simulink model "sim_closed_loop_with_identifiedmodel"  (R2024a)
settings: Solver=FixedStepAuto  StartTime=0.0  StopTime=10  FixedStep=1/fs  RelTol=1e-3
PostLoadFcn:
  | if any(exist('dsrtsu_mdlpostloadfcn', 'file') ~= 0), dsrtsu_mdlpostloadfcn('Execute', bdroot); end
InitFcn:
  | , if any(exist('rtifpga_mdlclblib', 'file') ~= 0), rtifpga_mdlclblib('Init', bdroot); end,
  | , if any(exist('dsmpb_private', 'file') ~= 0), dsmpb_private('dsmpb_mdlclblib', 'Init', bdroot); end,
values from neighbouring files (symbols this model uses):
  fcut = 2    [Fig09_compute_Xcorr_CLID.m]
  fs = 2000    [Fig09_compute_Xcorr_CLID.m]    (also in Fig10_compare_ID_closedloop.m)
  KdDMD = dlqr(Akdmd, Bkdmd, Qkdmd, 1)    [Fig09_compute_Xcorr_CLID.m]
  nuf = size(Bf,2)    [Fig09_compute_Xcorr_CLID.m]
  nxf = size(Af,1)    [Fig09_compute_Xcorr_CLID.m]
  sysID2 = sysID    [Fig09_compute_Xcorr_CLID.m]
  x0 = zeros(nzeta,1)    [Fig09_compute_Xcorr_CLID.m]
undefined symbols (not defined in the file or in its folder): Af, Bf
libraries: dspfdesign x1
PreSaveFcn:
  | , if any(exist('dsmpb_private', 'file') ~= 0), dsmpb_private('dsmpb_mdlclblib', 'PreSave', bdroot); end,
CloseFcn:
  | , if any(exist('dsmpb_private', 'file') ~= 0), dsmpb_private('dsmpb_mdlclblib', 'Close', bdroot); end,
settings Model: DSRTSU_INTERNAL_RTI_VER=570  DSRTSU_INTERNAL_RTI_TYPE=rti1202  RTICANMMDATA=struct('GeneralSetupData',struct('modelroot',['C:\Users\fthais\Desktop\Fernanda 03-25\Matlab - Simulink\10-07'],'generalsettings',struct('filesettings',struct('destfolder',struct('Name','RTICANMM_FILES','Check',1),'buildfolder',struct('Name','.','Check',1),'AbsDestfolder',struct('Name',['C:\Users\fthais\Desktop\Fernanda 03-25\Matlab - Simulink\10-07\RTICANMM_FILES']),'AbsBuildfolder',struct('Name',['C:\Users\fthais\Desktop\Fernanda 03-25\Matlab - Simulink\10-07']))),'options',struct('addpaths',1,'rmpaths',1,'addtrcexclusion',true,'cannavigator',struct('checkmonitoring',0),'show_usrtrc',0,'use_usrtrc',0),'advanced',struct('options',ones(1,100)),'MPSetup',{{}},'RTI',struct('Type','RTI1202','Ver','7.15','Date','02-Nov-2020'),'modelname','comm_beam','block','comm_beam'))  DSRTSU_INTERNAL_RTIFPGA=170  Creator=ADP-sletellier  LastModifiedBy=fertc
settings SolverCC: AlgebraicLoopSolver=TrustRegion
settings OptimizationCC: BlockReduction=off  ConditionallyExecuteInputs=off  OptimizeBlockIOStorage=off  BufferReuse=off  GlobalBufferReuse=off  ExpressionFolding=off  LocalBlockOutputs=off  OptimizeDataStoreBuffers=off  BusAssignmentInplaceUpdate=off
settings DebuggingCC: TasksWithSamePriorityMsg=none  UnconnectedInputMsg=warning  UnconnectedOutputMsg=warning  UnconnectedLineMsg=warning
settings HardwareCC: ProdBitPerPointer=32  ProdBitPerSizeT=32  ProdBitPerPtrDiffT=32  ProdLargestAtomicInteger=Integer  ProdEndianess=BigEndian  ProdWordSize=32  ProdLongLongMode=on  ProdHWDeviceType=Custom Processor->Custom  TargetIntDivRoundTo=Zero  TargetEndianess=BigEndian  TargetHWDeviceType=Custom Processor->Custom
settings ModelReferenceCC: EnableRefExpFcnMdlSchedulingChecks=on  EnableParallelModelReferenceBuilds=on
settings SFSimCC: MATLABDynamicMemAlloc=off
settings RTWCC: Description=dSPACE DS1202 Hardware Platform  SystemTargetFile=rti1202.tlc  GenCodeOnly=on  MakeCommand=make_rti  TemplateMakefile=rti1202.tmf  RTWVerbose=off  GPUComputeCapability=3.5
settings STFCustomTargetCC: TargetLangStandard=C89/C90 (ANSI)  ParMdlRefBuildCompliant=on  GRTInterface=off  UseToolchainInfoCompliant=off  SystemTargetFile=rti1202.tlc
settings GRTTargetCC: TargetLangStandard=C89/C90 (ANSI)  CompOptLevelCompliant=off  ConcurrentExecutionCompliant=off  CombineOutputUpdateFcns=off  MatFileLogging=off  CPPClassGenCompliant=off  UseToolchainInfoCompliant=off

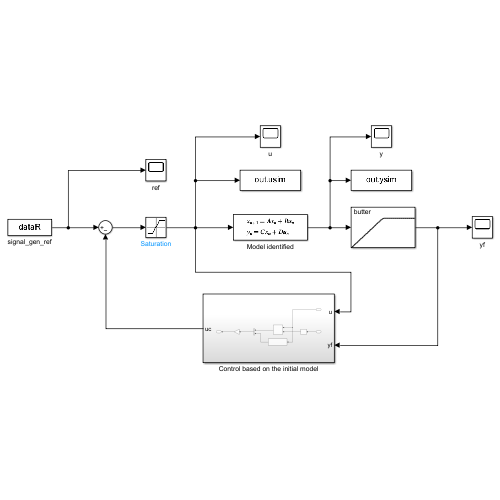
[thumbnail: Simulink's stored preview of the top-level diagram]
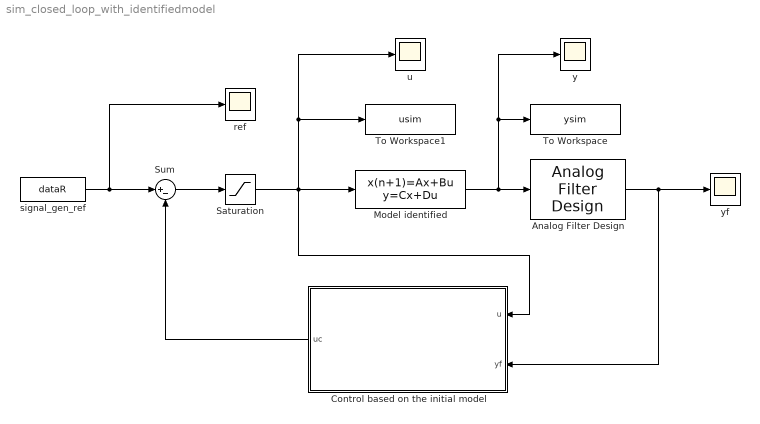
== system sim_closed_loop_with_identifiedmodel ==
  Analog Filter Design : dspfdesign/Analog Filter Design  method=Butterworth  filttype=Highpass  N=8  Wlo=2*pi*fcut  Whi=80  Rp=2  Rs=40
  Control based on the initial model : Subsystem
  Model identified : DiscreteStateSpace  A=sysID2.A  B=sysID2.B  C=sysID2.C  D=sysID2.D  SampleTime=1/fs
  Saturation : Saturate  UpperLimit=10  LowerLimit=-10
  Sum : Sum  Inputs=|+-
  To Workspace : ToWorkspace  VariableName=ysim  SaveFormat=Timeseries  SampleTime=-1
  To Workspace1 : ToWorkspace  VariableName=usim  SaveFormat=Timeseries  SampleTime=-1
  ref : Scope
  signal_gen_ref : FromWorkspace  VariableName=dataR  SampleTime=1/fs  Interpolate=off  OutputAfterFinalValue=Setting to zero
  u : Scope
  y : Scope
  yf : Scope
  wires:
  Analog Filter Design/1 -> yf/1, Control based on the initial model/2(yf)
  Saturation/1 -> Model identified/1, u/1, To Workspace1/1, Control based on the initial model/1(u)
  signal_gen_ref/1 -> ref/1, Sum/1
  Sum/1 -> Saturation/1
  Model identified/1 -> y/1, To Workspace/1, Analog Filter Design/1
  Control based on the initial model/1(uc) -> Sum/2

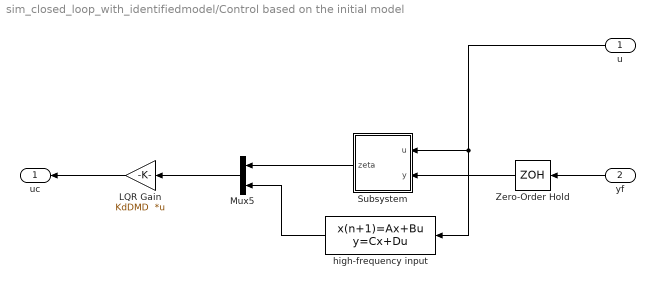
== system sim_closed_loop_with_identifiedmodel/Control based on the initial model ==
  u : Inport
  yf : Inport  Port=2
  LQR Gain : Gain  Gain=KdDMD  Multiplication=Matrix(K*u)
  Mux5 : Mux  Inputs=2
  Subsystem : Subsystem
  Zero-Order Hold : ZeroOrderHold  SampleTime=1/fs
  high-frequency input : DiscreteStateSpace  A=Af  B=Bf  C=eye(nxf)  D=zeros(nxf,nuf)  SampleTime=1/fs
  uc : Outport
  wires:
  Mux5/1 -> LQR Gain/1
  yf/1 -> Zero-Order Hold/1
  Subsystem/1(zeta) -> Mux5/1
  u/1 -> high-frequency input/1, Subsystem/1(u)
  high-frequency input/1 -> Mux5/2
  Zero-Order Hold/1 -> Subsystem/2(y)
  LQR Gain/1 -> uc/1

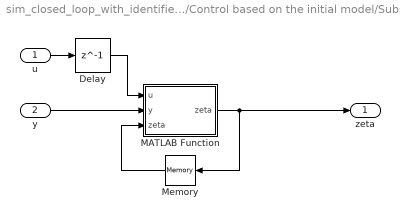
== system sim_closed_loop_with_identifiedmodel/Control based on the initial model/Subsystem ==
  u : Inport
  y : Inport  Port=2
  Delay : Delay  DelayLength=1  SampleTime=1/fs
  MATLAB Function : MATLAB Function  TreatAsAtomicUnit=on
  Memory : Memory  InitialCondition=x0
  zeta : Outport
  wires:
  MATLAB Function/1(zeta) -> Memory/1, zeta/1
  Delay/1 -> MATLAB Function/1(u)
  u/1 -> Delay/1
  Memory/1 -> MATLAB Function/3("zeta ")
  y/1 -> MATLAB Function/2(y)

== matlab function sim_closed_loop_with_identifiedmodel/Control based on the initial model/Subsystem/MATLAB Function ==
  data: u input; zeta output; y input; zeta input
function zeta = fcn(u,y,zeta)
nu = size(u,1); ny = size(y,1);
zeta = [ y; u; zeta(1:end - (ny+nu))];
